simulink model "PacketizedNetwork4Node"  (R2025b)
settings: Solver=FixedStepDiscrete  StartTime=0.0  StopTime=200000*Ts  FixedStep=Ts/6  RelTol=1e-3
InitFcn:
  | load networkParams;
  | Ts=1/1e7;
  | ALOHA = 1;
  | CSMA = 0;
  | CA = 1;
values from neighbouring files (symbols this model uses):
  L3payload = [0 0 0 1 0 0 0 0 1 1 1 0 ... (1040 elements, 1040x1)]    [networkParams.mat]
libraries: PacketizedNetworkLib x8, dspsigops x4, commchan3 x1, dspindex x1
Description:
  | This Simulink(R) Model simulates a 3-node wireless network.  Each node in the network has a physical layer and a data link layer of the OSI model.
settings Model: SimulationMode=accelerator  NumberOfSteps=100  Creator=The MathWorks, Inc.  LastModifiedBy=Sasith Induwara
settings SolverCC: AlgebraicLoopSolver=TrustRegion
settings DataIOCC: DSMLogging=off  ReturnWorkspaceOutputs=off
settings OptimizationCC: EfficientMapNaN2IntZero=off
settings DebuggingCC: UnconnectedInputMsg=warning  UnconnectedOutputMsg=warning  UnconnectedLineMsg=warning  ArithmeticOperatorsInVariantConditions=warning
settings HardwareCC: TargetBitPerPointer=64.0  TargetBitPerSizeT=64.0  TargetBitPerPtrDiffT=64.0  TargetLongLongMode=on  TargetIntDivRoundTo=Zero  TargetEndianess=LittleEndian  TargetWordSize=64.0  TargetHWDeviceType=MATLAB Host  ProdEqTarget=off
settings ModelReferenceCC: EnableRefExpFcnMdlSchedulingChecks=on
settings SFSimCC: SimUseLocalCustomCode=off  CustomCodeUndefinedFunction=UseInterfaceOnly
settings RTWCC: RTWUseLocalCustomCode=off  GPUComputeCapability=3.5
settings CodeAppCC: MaxIdLength=128.0  StateflowObjectComments=on
settings GRTTargetCC: TargetLangStandard=C89/C90 (ANSI)  CombineOutputUpdateFcns=off  GRTInterface=on
settings SimscapeCC: SimscapeNormalizeSystem=off

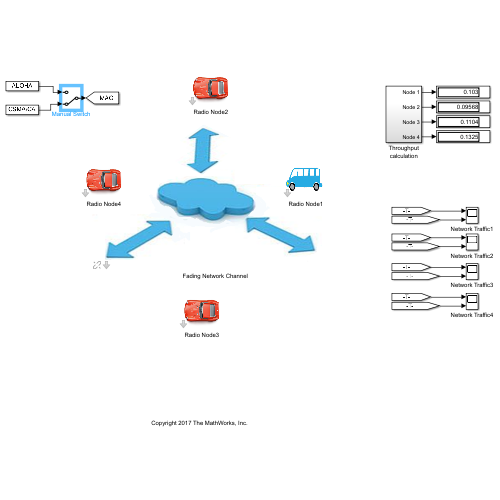
[thumbnail: Simulink's stored preview of the top-level diagram]
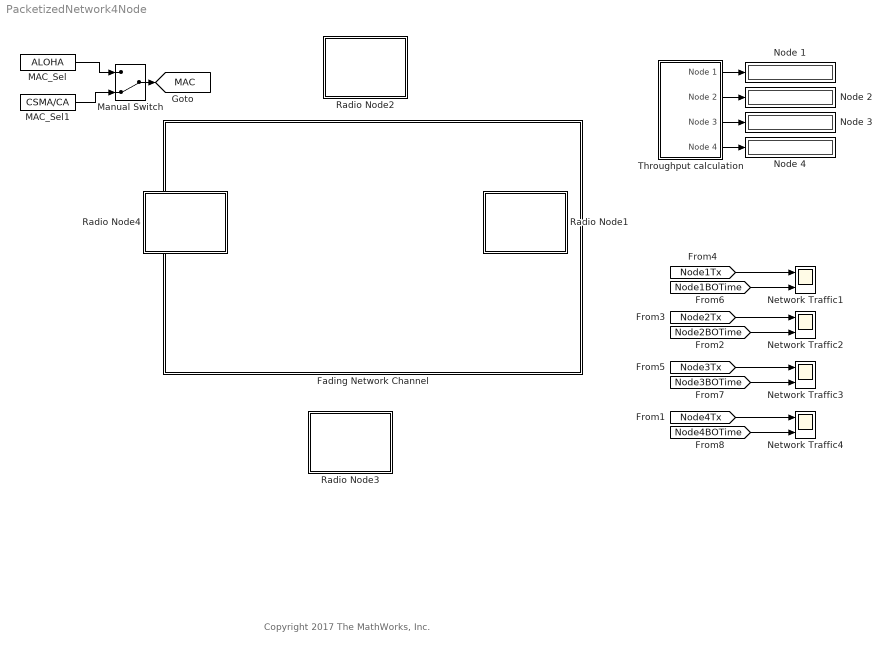
== system PacketizedNetwork4Node ==
  note: Copyright 2017 The MathWorks, Inc.
  Fading Network Channel : Subsystem  AncestorBlock=PacketizedNetworkLib/Fading Network Channel  mask(Radio Network){MDSN12=0.00000005/Ts, SNRN12=35, MDSN23=0.00000005/Ts, SNRN23=35, MDSN31=0.00000005/Ts, SNRN31=35}
      mask prompts: MDSN12 "Maximum Doppler Shift (Hz)"; SNRN12 "SNR of AWGN (Eb/No)"; MDSN23 "Maximum Doppler Shift (Hz)"; SNRN23 "SNR of AWGN (Eb/No)"; MDSN31 "Maximum Doppler Shift (Hz)"; SNRN31 "SNR of AWGN (Eb/No)"
      mask help: This model presents a radio network with Rayleigh fading channel between the transceiver nades.
      mask DialogControl ParameterGroupVar Prompt: Parameters for Channels
      mask DialogControl Container3 Prompt: Channel between Node 1 and Node 2
      mask DialogControl Container4 Prompt: Node 2 and Node 3
      mask DialogControl Container5 Prompt: Node 3 and Node 1
      mask Display: image('NetworkChannel.png');
  MAC_Sel : Constant  Value=ALOHA  OutDataTypeStr=boolean  SampleTime=Ts*8
  MAC_Sel1 : Constant  Value=CSMA/CA  OutDataTypeStr=boolean  SampleTime=Ts*8
  Manual Switch : ManualSwitch  CurrentSetting=0
  Network Traffic{1..4} (4 alike) : Scope  NumInputPorts=2
      Network Traffic1 settings: SampleTime=Ts/(2*3)  Title=Tx 1  ActiveDisplayYMinimum=-0.68347  ActiveDisplayYMaximum=0.68347  DataLoggingVariableName=ScopeData2
      Network Traffic2 settings: SampleTime=Ts/(2*3)  Title=Tx 2  ActiveDisplayYMinimum=-0.68347  ActiveDisplayYMaximum=0.68347  DataLoggingVariableName=ScopeData2
      Network Traffic3 settings: SampleTime=Ts/(2*3)  Title=Tx 3  ActiveDisplayYMinimum=-0.68347  ActiveDisplayYMaximum=0.68347
      Network Traffic4 settings: SampleTime=Ts/(2*3)  Title=Backoff 4  ActiveDisplayYMinimum=-47.875  ActiveDisplayYMaximum=420.875
  Node {1..4} (4 alike) : Display
  Radio Node1 : Subsystem  mask{NodeAddre=[0 0 0 0 0 0 0 1], DestAddre=[0 0 0 0 0 0 1 1], AckDestAddre=[0 0 0 0 0 1 0 0], lambda=1e3*8*Ts, pseed=10}
      mask prompts: NodeAddre "Node address:"; DestAddre "Data destination address:"; AckDestAddre "Ack destination address:"; lambda "Arrival rate (arrivals per slot time = 8*Ts):"; pseed "Random seed:"
      mask help:
      | The node address is the ID of the transceiver. The data destination address specifies the recipient of the data packets originating from this transceiver. The Ack destination address specifies the recipient of the acknowledgment packets originating from this transceiver.
      |
      | The lambda parameter regulates the frequency of generated data packets. Higher values specify longer packet interarrival times and therefore less frequent data frame generation.
      settings: NameChangeFcn=|
      | blkName = gcb;
      | set_param([gcb '/From'],'GotoTag',['Node' blkName(end) 'Rx']);
      | set_param([gcb '/Goto'],'GotoTag',['Node' blkName(end) 'Tx']);
      mask DialogControl Container2 Prompt: Parameters
      mask Display:
      | if contains(gcb, 'Node1')
      |   image('Car1.png');
      | else
      |   image('Car2.png');
      | end
  Radio Node2 : Subsystem  mask{NodeAddre=[0 0 0 0 0 0 1 0], DestAddre=[0 0 0 0 0 1 0 0], AckDestAddre=[0 0 0 0 0 0 1 1], lambda=1e3*8*Ts, pseed=13}
      mask prompts: NodeAddre "Node address:"; DestAddre "Data destination address:"; AckDestAddre "Ack destination address:"; lambda "Arrival rate (arrivals per slot time = 8*Ts):"; pseed "Random seed:"
      mask help:
      | The node address is the ID of the transceiver. The data destination address specifies the recipient of the data packets originating from this transceiver. The Ack destination address specifies the recipient of the acknowledgment packets originating from this transceiver.
      |
      | The lambda parameter regulates the frequency of generated data packets. Higher values specify longer packet interarrival times and therefore less frequent data frame generation.
      mask DialogControl Container2 Prompt: Parameters
      mask Display: image('Car2.png');
  Radio Node3 : Subsystem  mask{NodeAddre=[0 0 0 0 0 0 1 1], DestAddre=[0 0 0 0 0 0 1 0], AckDestAddre=[0 0 0 0 0 0 0 1], lambda=1e3*8*Ts, pseed=100}
      mask prompts: NodeAddre "Node address:"; DestAddre "Data destination address:"; AckDestAddre "Ack destination address:"; lambda "Arrival rate (arrivals per slot time = 8*Ts):"; pseed "Random seed:"
      mask help:
      | The node address is the ID of the transceiver. The data destination address specifies the recipient of the data packets originating from this transceiver. The Ack destination address specifies the recipient of the acknowledgment packets originating from this transceiver.
      |
      | The lambda parameter regulates the frequency of generated data packets. Higher values specify longer packet interarrival times and therefore less frequent data frame generation.
      mask Display: image('Car2.png');
  Radio Node4 : Subsystem  mask{NodeAddre=[0 0 0 0 0 1 0 0], DestAddre=[0 0 0 0 0 0 0 1], AckDestAddre=[0 0 0 0 0 0 1 0], lambda=1e3*8*Ts, pseed=42}
      mask prompts: NodeAddre "Node address:"; DestAddre "Data destination address:"; AckDestAddre "Ack destination address:"; lambda "Arrival rate (arrivals per slot time = 8*Ts):"; pseed "Random seed:"
      mask help:
      | The node address is the ID of the transceiver. The data destination address specifies the recipient of the data packets originating from this transceiver. The Ack destination address specifies the recipient of the acknowledgment packets originating from this transceiver.
      |
      | The lambda parameter regulates the frequency of generated data packets. Higher values specify longer packet interarrival times and therefore less frequent data frame generation.
      mask Display: image('Car2.png');
  Throughput calculation : Subsystem
  tag scope: MAC=global
  wires:
  MAC_Sel/1 -> Manual Switch/1
  MAC_Sel1/1 -> Manual Switch/2
  Manual Switch/1 -> [MAC]
  [Node1Tx] -> Network Traffic1/1
  [Node1BOTime] -> Network Traffic1/2
  [Node2Tx] -> Network Traffic2/1
  [Node2BOTime] -> Network Traffic2/2
  [Node3Tx] -> Network Traffic3/1
  [Node3BOTime] -> Network Traffic3/2
  Throughput calculation/1(Node 1) -> Node 1/1
  Throughput calculation/2(Node 2) -> Node 2/1
  Throughput calculation/3(Node 3) -> Node 3/1
  Throughput calculation/4(Node 4) -> Node 4/1
  [Node4Tx] -> Network Traffic4/1
  [Node4BOTime] -> Network Traffic4/2

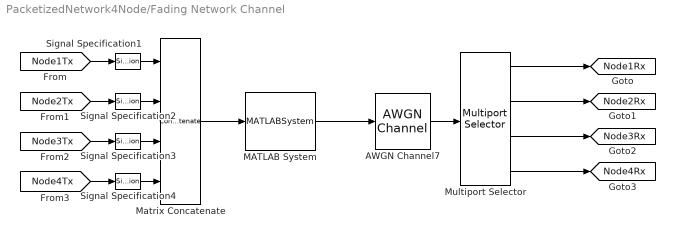
== system PacketizedNetwork4Node/Fading Network Channel ==
  AWGN Channel7 : commchan3/AWGN Channel  LegacyMode=off  NoiseMethod="Signal to noise ratio  (Eb/No)"  noiseMode="Signal to noise ratio  (SNR)"  EbNo=[SNRN12, SNRN23, SNRN31, SNRN31]  EsNo=10  SNR=10  BitsPerSymbol=2  SignalPower=0.1634  SpecifySymbolPeriod=off  SamplesPerSymbol=1  SymbolPeriod=Ts  VarianceSource=Parameter  Variance=1  RandomStream=mt19937ar with seed  Seed=67  SimulateUsing=Code generation
  MATLAB System : MATLABSystem  System=NetworkChannel  SampleRateSource=Input port  SampleRate=[ 1e3, 2e3, 3e3 ]  PathDelays={[0 0.3*Ts], [0 0.3*Ts], [0 0.3*Ts]; [0 0.3*Ts], [0 0.3*Ts], [0 0.3*Ts]; [0 0.3*Ts], [0 0.3*Ts], [0 0.3*Ts]; [0 0.3*Ts], [0 0.3*Ts], [0 0.3*Ts]}  AveragePathGains={[0 -6],[0 -6] ,[0 -6]; [0 -6],[0 -6] ,[0 -6]; [0 -6],[0 -6] ,[0 -6]; [0 -6],[0 -6] ,[0 -6];}  MaximumDopplerShift=repmat(0.00000005/Ts, 4, 3)  SimulateUsing=Code generation
      mask Type: NetworkChannel
  Matrix Concatenate : Concatenate  NumInputs=4  Mode=Multidimensional array  ConcatenateDimension=2
  Multiport Selector : dspindex/Multiport Selector  rowsOrCols=Columns  idxCellArray=num2cell(1:4)  idxErrMode=Clip Index
  Signal Specification{1..4} (4 alike) : SignalSpecification  Dimensions=1
  tag scope: Node1Rx=global, Node2Rx=global, Node3Rx=global, Node4Rx=global
  wires:
  MATLAB System/1 -> AWGN Channel7/1
  AWGN Channel7/1 -> Multiport Selector/1
  Multiport Selector/3 -> [Node3Rx]
  Multiport Selector/2 -> [Node2Rx]
  Multiport Selector/1 -> [Node1Rx]
  Signal Specification3/1 -> Matrix Concatenate/3
  Signal Specification2/1 -> Matrix Concatenate/2
  Signal Specification1/1 -> Matrix Concatenate/1
  Matrix Concatenate/1 -> MATLAB System/1
  [Node3Tx] -> Signal Specification3/1
  [Node2Tx] -> Signal Specification2/1
  [Node1Tx] -> Signal Specification1/1
  [Node4Tx] -> Signal Specification4/1
  Signal Specification4/1 -> Matrix Concatenate/4
  Multiport Selector/4 -> [Node4Rx]

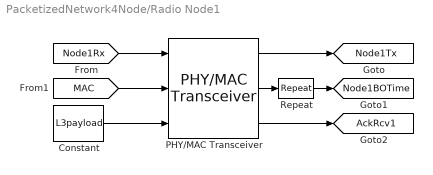
== system PacketizedNetwork4Node/Radio Node1 ==
  Constant : Constant  Value=L3payload
  PHY/MAC Transceiver : PacketizedNetworkLib/PHY//MAC Transceiver  SystemSampleTime=-1  VariantActivationTime=update diagram  EmptyChoice=off  PassThrough=off  PassThroughVariantControl=(default)  EmptyChoiceVariantControl=(default)  AllowFlexibleInterface=on  Latency=0  AutoFrameSizeCalculation=off
  Repeat : dspsigops/Repeat  FactorSource=Dialog parameter  N=48  Nmax=16  InputProcessing=Columns as channels (frame based)  RateOptions=Allow multirate processing  ic=0  mode=Unused parameter value
  tag scope: AckRcv1=global, Node1BOTime=global, Node1Tx=global
  wires:
  [MAC] -> PHY/MAC Transceiver/2
  PHY/MAC Transceiver/2 -> Repeat/1
  PHY/MAC Transceiver/1 -> [Node1Tx]
  [Node1Rx] -> PHY/MAC Transceiver/1
  Constant/1 -> PHY/MAC Transceiver/3
  Repeat/1 -> [Node1BOTime]
  PHY/MAC Transceiver/3 -> [AckRcv1]

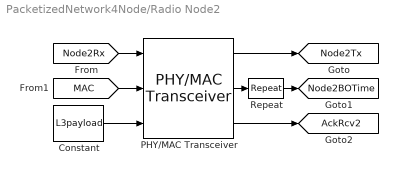
== system PacketizedNetwork4Node/Radio Node2 ==
  Constant : Constant  Value=L3payload
  PHY/MAC Transceiver : PacketizedNetworkLib/PHY//MAC Transceiver  SystemSampleTime=-1  VariantActivationTime=update diagram  EmptyChoice=off  PassThrough=off  PassThroughVariantControl=(default)  EmptyChoiceVariantControl=(default)  AllowFlexibleInterface=on  Latency=0  AutoFrameSizeCalculation=off
  Repeat : dspsigops/Repeat  FactorSource=Dialog parameter  N=48  Nmax=16  InputProcessing=Columns as channels (frame based)  RateOptions=Allow multirate processing  ic=0  mode=Unused parameter value
  tag scope: AckRcv2=global, Node2BOTime=global, Node2Tx=global
  wires:
  [Node2Rx] -> PHY/MAC Transceiver/1
  PHY/MAC Transceiver/1 -> [Node2Tx]
  [MAC] -> PHY/MAC Transceiver/2
  PHY/MAC Transceiver/2 -> Repeat/1
  Constant/1 -> PHY/MAC Transceiver/3
  Repeat/1 -> [Node2BOTime]
  PHY/MAC Transceiver/3 -> [AckRcv2]

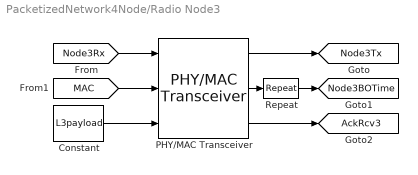
== system PacketizedNetwork4Node/Radio Node3 ==
  Constant : Constant  Value=L3payload
  PHY/MAC Transceiver : PacketizedNetworkLib/PHY//MAC Transceiver  SystemSampleTime=-1  VariantActivationTime=update diagram  EmptyChoice=off  PassThrough=off  PassThroughVariantControl=(default)  EmptyChoiceVariantControl=(default)  AllowFlexibleInterface=on  Latency=0  AutoFrameSizeCalculation=off
  Repeat : dspsigops/Repeat  FactorSource=Dialog parameter  N=48  Nmax=16  InputProcessing=Columns as channels (frame based)  RateOptions=Allow multirate processing  ic=0  mode=Unused parameter value
  tag scope: AckRcv3=global, Node3BOTime=global, Node3Tx=global
  wires:
  [Node3Rx] -> PHY/MAC Transceiver/1
  PHY/MAC Transceiver/1 -> [Node3Tx]
  [MAC] -> PHY/MAC Transceiver/2
  PHY/MAC Transceiver/2 -> Repeat/1
  Constant/1 -> PHY/MAC Transceiver/3
  Repeat/1 -> [Node3BOTime]
  PHY/MAC Transceiver/3 -> [AckRcv3]

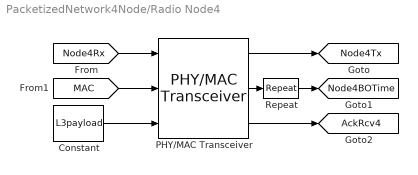
== system PacketizedNetwork4Node/Radio Node4 ==
  Constant : Constant  Value=L3payload
  PHY/MAC Transceiver : PacketizedNetworkLib/PHY//MAC Transceiver  SystemSampleTime=-1  VariantActivationTime=update diagram  EmptyChoice=off  PassThrough=off  PassThroughVariantControl=(default)  EmptyChoiceVariantControl=(default)  AllowFlexibleInterface=on  Latency=0  AutoFrameSizeCalculation=off
  Repeat : dspsigops/Repeat  FactorSource=Dialog parameter  N=48  Nmax=16  InputProcessing=Columns as channels (frame based)  RateOptions=Allow multirate processing  ic=0  mode=Unused parameter value
  tag scope: AckRcv4=global, Node4BOTime=global, Node4Tx=global
  wires:
  [Node4Rx] -> PHY/MAC Transceiver/1
  PHY/MAC Transceiver/1 -> [Node4Tx]
  [MAC] -> PHY/MAC Transceiver/2
  PHY/MAC Transceiver/2 -> Repeat/1
  Constant/1 -> PHY/MAC Transceiver/3
  Repeat/1 -> [Node4BOTime]
  PHY/MAC Transceiver/3 -> [AckRcv4]

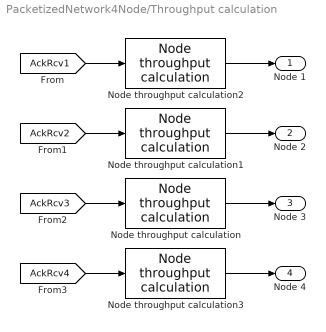
== system PacketizedNetwork4Node/Throughput calculation ==
  Node throughput calculation{,1..3} (4 alike) : PacketizedNetworkLib/Node throughput calculation  SystemSampleTime=-1  VariantActivationTime=update diagram  EmptyChoice=off  PassThrough=off  PassThroughVariantControl=(default)  EmptyChoiceVariantControl=(default)  AllowFlexibleInterface=on  Latency=0  AutoFrameSizeCalculation=off
  Node 1 : Outport  VectorParamsAs1DForOutWhenUnconnected=off
  Node 2 : Outport  Port=2  VectorParamsAs1DForOutWhenUnconnected=off
  Node 3 : Outport  Port=3  VectorParamsAs1DForOutWhenUnconnected=off
  Node 4 : Outport  Port=4  VectorParamsAs1DForOutWhenUnconnected=off
  wires:
  [AckRcv1] -> Node throughput calculation2/1
  [AckRcv2] -> Node throughput calculation1/1
  Node throughput calculation1/1 -> Node 2/1
  [AckRcv3] -> Node throughput calculation/1
  Node throughput calculation/1 -> Node 3/1
  Node throughput calculation2/1 -> Node 1/1
  [AckRcv4] -> Node throughput calculation3/1
  Node throughput calculation3/1 -> Node 4/1
